simulink model "tutorial35_imu"  (R2025a)
settings: Solver=VariableStepAuto  StartTime=0.0  StopTime=10.0  RelTol=1e-3
settings Model: Creator=xing2  LastModifiedBy=xing2

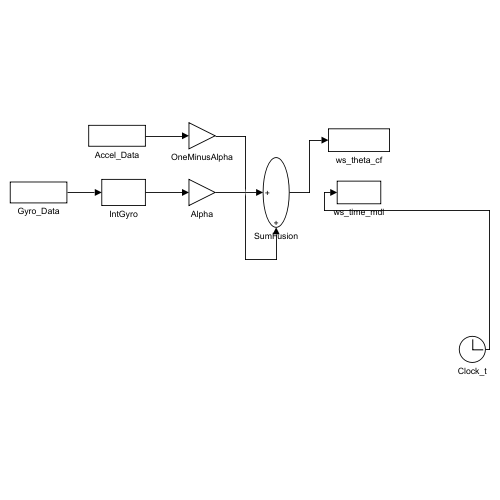
[thumbnail: Simulink's stored preview of the top-level diagram]
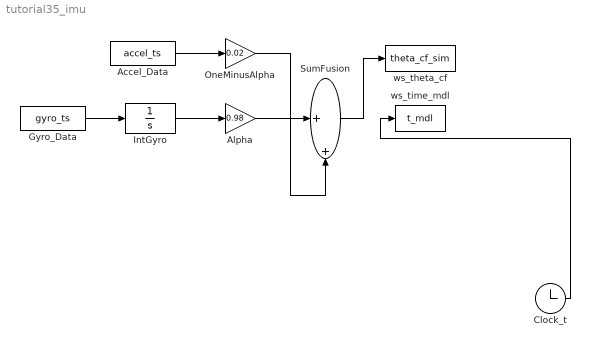
== system tutorial35_imu ==
  Accel_Data : FromWorkspace  VariableName=accel_ts
  Alpha : Gain  Gain=0.98
  Clock_t : Clock
  Gyro_Data : FromWorkspace  VariableName=gyro_ts
  IntGyro : Integrator
  OneMinusAlpha : Gain  Gain=0.02
  SumFusion : Sum  Inputs=|++
  ws_theta_cf : ToWorkspace  VariableName=theta_cf_sim  SaveFormat=Timeseries  SampleTime=-1
  ws_time_mdl : ToWorkspace  VariableName=t_mdl  SaveFormat=Timeseries  SampleTime=-1
  wires:
  Accel_Data/1 -> OneMinusAlpha/1
  Gyro_Data/1 -> IntGyro/1
  Alpha/1 -> SumFusion/1
  IntGyro/1 -> Alpha/1
  OneMinusAlpha/1 -> SumFusion/2
  SumFusion/1 -> ws_theta_cf/1
  Clock_t/1 -> ws_time_mdl/1
